simulink model "sns_tutorial8_twin"  (R2025a)
settings: Solver=ode1  StartTime=0.0  StopTime=5  FixedStep=1e-3  RelTol=1e-3
libraries: SNS_Deng_Library x2, SNS_Library x2
settings Model: Creator=Ben Bolen  LastModifiedBy=Ben Bolen
settings DataIOCC: SignalLoggingName=sigs

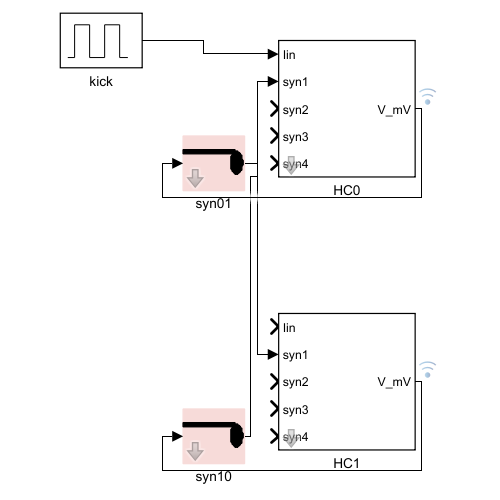
[thumbnail: Simulink's stored preview of the top-level diagram]
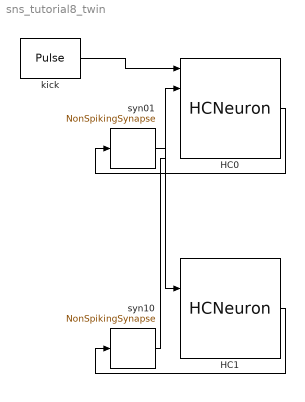
== system sns_tutorial8_twin ==
  HC0 : SNS_Deng_Library/HCNeuron  Cm=5  Gm=1  Vrest=-60  GNa=1.048507073  ENa=50  Sm=0.05  Em=-40  Km=1  Sh=-0.05  Eh=-60  Kh=0.5  hPowExp=1  tauH=300  h0=0.6666666667
  HC1 : SNS_Deng_Library/HCNeuron  Cm=5  Gm=1  Vrest=-60  GNa=1.048507073  ENa=50  Sm=0.05  Em=-40  Km=1  Sh=-0.05  Eh=-60  Kh=0.5  hPowExp=1  tauH=300  h0=0.6666666667
  kick : DiscretePulseGenerator  PulseType=Time based  Period=50  PulseWidth=0.002  PhaseDelay=0.001
  syn01 : SNS_Library/NonSpikingSynapse  gmax=0.1724044667  Esyn=-180  ThrPre=-60  SlopePre=20
  syn10 : SNS_Library/NonSpikingSynapse  gmax=0.1724044667  Esyn=-180  ThrPre=-60  SlopePre=20
  wires:
  kick/1 -> HC0/1
  HC0/1 -> syn01/1
  syn01/1 -> HC1/2
  HC1/1 -> syn10/1
  syn10/1 -> HC0/2
